simulink model "simWECS_2019a_LUT"  (R2019a)
settings: Solver=FixedStepAuto  StartTime=0.0  StopTime=40*DT  FixedStep=DT  RelTol=1e-3
values from neighbouring files (symbols this model uses):
  Cq = 0.0 0.0 0.0 0.0 0.0 0.0 0.0 0.0 0.0 0.0 0.0 0.0 0.0 0.0 0.0 0.0 0.0 0.0 0.0 0.0 0.0 0.0 0.0 0.0 0.0 0.0 0.0 0.0 0.0 0.0 0.0 0.0 0.0 0.0 0.0 0.0 0.0 0.0 0.0 0.0 0.0 0.0 0.0 0.0 0.0 0.0 0.0 0.0 0.0 0.0 0.0 0.0 0.0 0.0 0.0 0.0 0.0 0.0 0.0 0.0 0.0 0.0 0.0 0.0 0.0 0.0 0.0 0.0 0.0 0.0 0.0 0.0 0.0 0.0 0.0 0.0 0.0 0.0 0.0 0.0 0.0 0.0 0.0 0.0 0.0 0.0 0.0 0.0 0.0 0.0 0.0 0.0 0.0 0.0 0.0 0.0 0.0 0.0 0.0 0.0    [DD_test.sldd]    (also in testOutList.m = saveVarsMat.Cq)
  Ct = 0.0 0.0 0.0 0.0 0.0 0.0 0.0 0.0 0.0 0.0 0.0 0.0 0.0 0.0 0.0 0.0 0.0 0.0 0.0 0.0 0.0 0.0 0.0 0.0 0.0 0.0 0.0 0.0 0.0 0.0 0.0 0.0 0.0 0.0 0.0 0.0 0.0 0.0 0.0 0.0 0.0 0.0 0.0 0.0 0.0 0.0 0.0 0.0 0.0 0.0 0.0 0.0 0.0 0.0 0.0 0.0 0.0 0.0 0.0 0.0 0.0 0.0 0.0 0.0 0.0 0.0 0.0 0.0 0.0 0.0 0.0 0.0 0.0 0.0 0.0 0.0 0.0 0.0 0.0 0.0 0.0 0.0 0.0 0.0 0.0 0.0 0.0 0.0 0.0 0.0 0.0 0.0 0.0 0.0 0.0 0.0 0.0 0.0 0.0 0.0    [DD_test.sldd]    (also in testOutList.m = saveVarsMat.Ct)
  Drivetrain = struct    [dataDLR.m]
  DT = 0.008    [dataDLR.m]    (also in generateReport.m; initLPVParam.m; initWorkspace.m; runCalculateEvalCriteria.m)
  Lin_points : value not decoded    [DD_test.sldd]
  mu_old = zeros(2*N*nu,1)    [testCtrl.m]
  Ng = 97    [dataDLR.m]    (also in testCtrl.m)
  omegabar = interp1(Lin_points.V,Lin_points.RSpeed,Vbar,'spline')    [testCtrl.m]
  rho = 1.225    [DD_test.sldd]    (also in dataDLR.m; testOutList.m; testqLPV.m)
  tau_g = 0.01    [testCtrl.m]
  U = zeros(2*N,1)    [testCtrl.m]
  xk = Xk(nxa+1:2*nxa)    [testCtrl.m]
  Xko = kron(ones(N,1),xk)    [testCtrl.m]
undefined symbols (not defined in the file or in its folder): R, Rotor_Lambda, Rotor_Lamda, Rotor_Pitch
settings Model: ExtModeTrigMode=oneshot  ExtModeArmWhenConnect=off  Creator=Hazim Namik  LastModifiedBy=bs
settings DataIOCC: LimitDataPoints=on  SaveFormat=Array  ReturnWorkspaceOutputs=off
settings OptimizationCC: BlockReduction=off  BooleanDataType=off  LifeSpan=inf
settings DebuggingCC: SaveWithParameterizedLinksMsg=none  UnderspecifiedInitializationDetection=Classic  MergeDetectMultiDrivingBlocksExec=none  SignalResolutionControl=TryResolveAllWithWarning  SFUnexpectedBacktrackingDiag=warning  SFNoUnconditionalDefaultTransitionDiag=warning  SFExecutionAtInitializationDiag=none  ArithmeticOperatorsInVariantConditions=warning
settings HardwareCC: ProdBitPerPointer=32  ProdBitPerSizeT=32  ProdBitPerPtrDiffT=32  ProdLargestAtomicFloat=None  ProdIntDivRoundTo=Undefined  ProdEndianess=Unspecified  ProdWordSize=32  ProdHWDeviceType=32-bit Generic  TargetUnknown=on
settings ModelReferenceCC: PropagateSignalLabelsOutOfModel=off
settings SFSimCC: SimUseLocalCustomCode=off
settings RTWCC: RTWUseLocalCustomCode=off
settings CodeAppCC: StateflowObjectComments=on
settings GRTTargetCC: TargetLangStandard=C89/C90 (ANSI)  GeneratePreprocessorConditionals=Disable all
settings ConfigComp: CovMetricSettings=dw  CovHtmlReporting=on  CovSaveCumulativeToWorkspaceVar=on  CovSaveSingleToWorkspaceVar=on  CovExternalEMLEnable=off

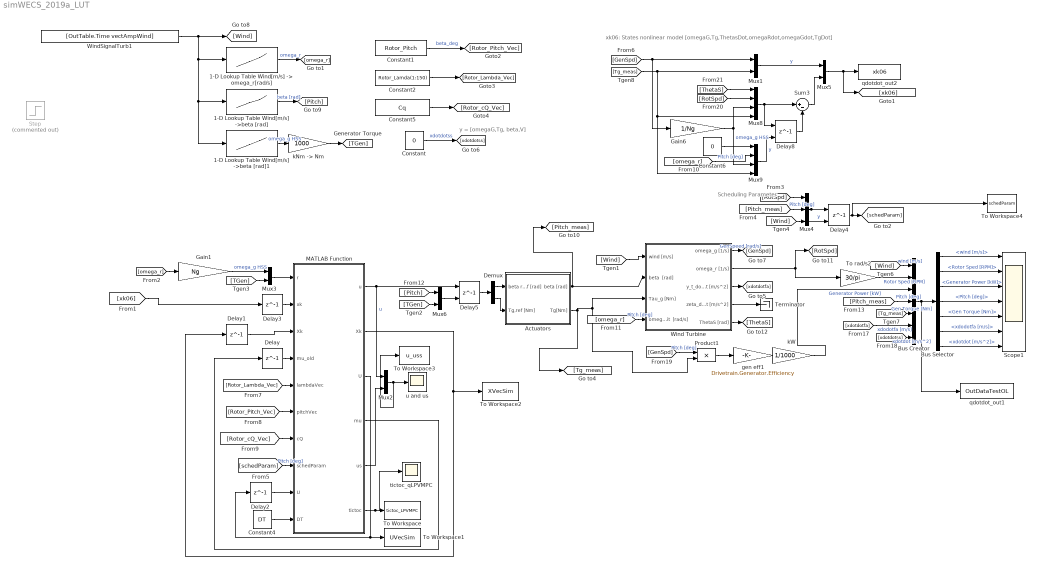
== system simWECS_2019a_LUT ==
  note: Scheduling Parameter
  note: xk06: States nonlinear model [omegaG,Tg,ThetasDot,omegaRdot,omegaGdot,TgDot]
  note: y = [omegaG,Tg, beta,V]
  "1-D Lookup Table Wind[m/s] -> omega_r[rad/s]" : Lookup_n-D  NumberOfTableDimensions=1  BreakpointsForDimension1=Lin_points.V  BreakpointsForDimension2=Rotor_Lambda  Table=Lin_points.RSpeed  InternalRulePriority=Speed  RndMeth=Simplest  InputSameDT=on
  1-D Lookup Table Wind[m/s] ->beta [rad] : Lookup_n-D  NumberOfTableDimensions=1  BreakpointsForDimension1=Lin_points.V  BreakpointsForDimension2=Rotor_Lambda  Table=Lin_points.Pitch  InternalRulePriority=Speed  RndMeth=Simplest  InputSameDT=on
  1-D Lookup Table Wind[m/s] ->beta [rad]1 : Lookup_n-D  NumberOfTableDimensions=1  BreakpointsForDimension1=Lin_points.V  BreakpointsForDimension2=Rotor_Lambda  Table=Lin_points.Torque  InternalRulePriority=Speed  RndMeth=Simplest  InputSameDT=on
  Actuators : Subsystem
  Bus Creator : BusCreator  Inputs=7
  Bus Selector : BusSelector  OutputSignals=wind [m/s],Rotor Sped [RPM],Generator Power [kW],Pitch [deg],Gen Torque [Nm],xdodotfa [m/s],xdotdot [m/s^2]
  Constant : Constant  Value=0
  Constant1 : Constant  Value=Rotor_Pitch
  Constant2 : Constant  Value=Rotor_Lamda(1:150)
  Constant4 : Constant  Value=DT
  Constant5 : Constant  Value=Cq
  Constant6 : Constant  Value=0
  Delay : Delay  DelayLength=1  InitialCondition=mu_old
  Delay1 : Delay  DelayLength=1  InitialCondition=Xko
  Delay2 : Delay  DelayLength=1  InitialCondition=U
  Delay3 : Delay  DelayLength=1  InitialCondition=xk
  Delay4 : Delay  DelayLength=1  InitialConditionSource=Input port  InitialCondition=[0,omegabar]
      settings: InputPortMap=u0,p4
  Delay5 : Delay  DelayLength=1  InitialConditionSource=Input port  InitialCondition=[0,omegabar]
      settings: InputPortMap=u0,p4
  Delay8 : Delay  DelayLength=1  InitialConditionSource=Input port  InitialCondition=[0,omegabar]
      settings: InputPortMap=u0,p4
  Demux : Demux  Outputs=2
  Gain1 : Gain  Gain=Ng
  Gain6 : Gain  Gain=1/Ng
  MATLAB Function : MATLAB Function  TreatAsAtomicUnit=on
  Mux{1..3,5..6} (5 alike) : Mux  Inputs=2
  Mux4 : Mux  Inputs=3
  Mux8 : Mux
  Mux9 : Mux
  Product1 : Product  RndMeth=Zero
  Scope1 : Scope  NumInputPorts=7
      settings: Tag=Scope
  Step : Step  Commented=on  Time=5  Before=11  After=12  SampleTime=0
  Sum3 : Sum  Inputs=|+-
  Terminator : Terminator
  To Workspace : ToWorkspace  VariableName=tictoc_LPVMPC  SaveFormat=Timeseries  SampleTime=-1
  To Workspace1 : ToWorkspace  VariableName=UVecSim  SampleTime=-1
  To Workspace2 : ToWorkspace  VariableName=XVecSim  SampleTime=-1
  To Workspace3 : ToWorkspace  VariableName=u_uss  SampleTime=-1
      settings: Save2DSignal=2-D array (concatenate along first dimension)
  To Workspace4 : ToWorkspace  VariableName=schedParam  SampleTime=-1
      settings: Save2DSignal=2-D array (concatenate along first dimension)
  To rad/s2 : Gain  Gain=30/pi
  Wind Turbine : Subsystem
  WindSignalTurb1 : FromWorkspace  VariableName=[OutTable.Time vectAmpWind]  SampleTime=DT  OutputAfterFinalValue=Holding final value
  gen eff1 : Gain  Gain=Drivetrain.Generator.Efficiency
  "kNm -> Nm" : Gain  Gain=1000
  kW : Gain  Gain=1/1000
  qdotdot_out1 : ToWorkspace  VariableName=OutDataTestOL  SampleTime=-1
  qdotdot_out2 : ToWorkspace  VariableName=xk06  SampleTime=-1
  tictoc_qLPVMPC : Scope
  u and us : Scope
  wires:
  MATLAB Function/5(us) -> Mux2/2
  1-D Lookup Table Wind[m/s] ->beta [rad]1/1 -> "kNm -> Nm"/1  "omega_g HSS"
  MATLAB Function/6(tictoc) -> tictoc_qLPVMPC/1, To Workspace/1
  "1-D Lookup Table Wind[m/s] -> omega_r[rad/s]"/1 -> [omega_r]  "omega_r"
  Delay/1 -> MATLAB Function/4(mu_old)
  Delay1/1 -> MATLAB Function/3("Xk ")
  Mux2/1 -> u and us/1, To Workspace3/1
  MATLAB Function/1(u) -> Delay5/1, Mux2/1  "u"
  MATLAB Function/4(mu) -> Delay/1
  1-D Lookup Table Wind[m/s] ->beta [rad]/1 -> [Pitch]  "beta [rad]"
  Constant2/1 -> [Rotor_Lambda_Vec]
  Constant1/1 -> [Rotor_Pitch_Vec]  "beta_deg"
  Constant5/1 -> [Rotor_cQ_Vec]
  WindSignalTurb1/1 -> 1-D Lookup Table Wind[m/s] ->beta [rad]1/1, 1-D Lookup Table Wind[m/s] ->beta [rad]/1, "1-D Lookup Table Wind[m/s] -> omega_r[rad/s]"/1, [Wind]
  "kNm -> Nm"/1 -> [TGen]
  [Rotor_Lambda_Vec] -> MATLAB Function/5(lambdaVec)
  [Rotor_Pitch_Vec] -> MATLAB Function/6(pitchVec)
  [Rotor_cQ_Vec] -> MATLAB Function/7(cQ)
  Bus Selector/6 -> Scope1/6  "<xdodotfa [m/s]>"
  Actuators/1(beta [rad]) -> [Pitch_meas], Wind Turbine/2(beta  [rad])
  To rad/s2/1 -> Bus Creator/2  "Rotor Sped [RPM]"
  Bus Selector/5 -> Scope1/5  "<Gen Torque [Nm]>"
  [GenSpd] -> Product1/1  "Pitch [deg]"
  [Tg_meas] -> Bus Creator/5  "Gen Torque [Nm]"
  [Wind] -> Wind Turbine/1(wind [m/s])
  Product1/1 -> gen eff1/1
  [xdotdotfa] -> Bus Creator/6  "xdodotfa [m/s]"
  [Pitch_meas] -> Bus Creator/4  "Pitch [deg]"
  Wind Turbine/4(zeta_dotdot [m/s^2]) -> Terminator/1
  Wind Turbine/2(omega_r [1/s]) -> To rad/s2/1, [RotSpd]
  [xdotdotss] -> Bus Creator/7  "xdotdot [m/s^2]"
  Constant/1 -> [xdotdotss]  "xdotdotss"
  Wind Turbine/1(omega_g [1/s]) -> [GenSpd]  "GenSpeed [rad/s]"
  [Wind] -> Bus Creator/1  "wind [m/s]"
  kW/1 -> Bus Creator/3  "Generator Power [kW]"
  Actuators/2(Tg[Nm]) -> [Tg_meas], Product1/2, Wind Turbine/3(Tau_g [Nm])
  Bus Creator/1 -> Bus Selector/1, qdotdot_out1/1
  Wind Turbine/3(y_t_dotdot [m/s^2]) -> [xdotdotfa]
  gen eff1/1 -> kW/1
  Wind Turbine/5(ThetaS [rad]) -> [ThetaS]
  Bus Selector/7 -> Scope1/7  "<xdotdot [m/s^2]>"
  Bus Selector/4 -> Scope1/4  "<Pitch [deg]>"
  Bus Selector/3 -> Scope1/3  "<Generator Power [kW]>"
  Bus Selector/2 -> Scope1/2  "<Rotor Sped [RPM]>"
  Bus Selector/1 -> Scope1/1  "<wind [m/s]>"
  [xk06] -> Delay3/1
  Delay2/1 -> MATLAB Function/9("U ")
  MATLAB Function/3(U) -> To Workspace1/1, Delay2/1
  [RotSpd] -> Mux4/1
  [Pitch_meas] -> Mux4/2  "Pitch [deg]"
  [Wind] -> Mux4/3
  [schedParam] -> MATLAB Function/8(schedParam)  "Pitch [deg]"
  Constant4/1 -> MATLAB Function/10(DT)
  Mux3/1 -> MATLAB Function/1(r)
  [omega_r] -> Gain1/1
  [TGen] -> Mux3/2
  Delay3/1 -> MATLAB Function/2(xk)
  MATLAB Function/2(Xk) -> To Workspace2/1, Delay1/1
  Demux/2 -> Actuators/2(Tg,ref [Nm])
  Demux/1 -> Actuators/1(beta ref [rad])
  [omega_r] -> Mux9/2  "Pitch [deg]"
  Constant6/1 -> Mux9/1
  Delay8/1 -> Sum3/2
  [ThetaS] -> Mux8/1
  Mux8/1 -> Sum3/1, Delay8/1
  [Tg_meas] -> Mux9/4, Mux8/4, Mux1/2
  Mux1/1 -> Mux5/1  "y"
  Mux9/1 -> Delay8/2  "y"
  [GenSpd] -> Gain6/1, Mux1/1
  [RotSpd] -> Mux8/2
  Gain6/1 -> Mux8/3, Mux9/3  "omega_g HSS"
  Mux5/1 -> [xk06], qdotdot_out2/1
  Sum3/1 -> Mux5/2
  Gain1/1 -> Mux3/1  "omega_g HSS"
  Delay4/1 -> To Workspace4/1, [schedParam]
  Mux4/1 -> Delay4/2, Delay4/1  "y"
  [Pitch] -> Mux6/1
  [TGen] -> Mux6/2
  Mux6/1 -> Delay5/2
  Delay5/1 -> Demux/1
  [omega_r] -> Wind Turbine/4(omega_r_init  [rad/s])  "Pitch [deg]"

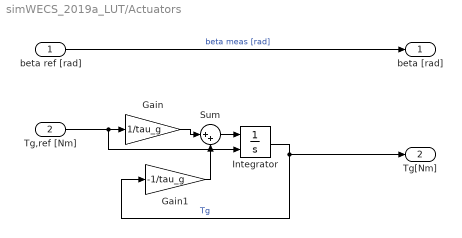
== system simWECS_2019a_LUT/Actuators ==
  beta ref [rad] : Inport
  Tg,ref [Nm] : Inport  Port=2
  Gain : Gain  Gain=1/tau_g
  Gain1 : Gain  Gain=-1/tau_g
  Integrator : Integrator  InitialConditionSource=external
  Sum : Sum  Inputs=|++
  beta [rad] : Outport
  Tg[Nm] : Outport  Port=2
  wires:
  Tg,ref [Nm]/1 -> Gain/1, Integrator/2
  Integrator/1 -> Tg[Nm]/1, Gain1/1  "Tg"
  beta ref [rad]/1 -> beta [rad]/1  "beta meas [rad]"
  Gain/1 -> Sum/1
  Sum/1 -> Integrator/1
  Gain1/1 -> Sum/2

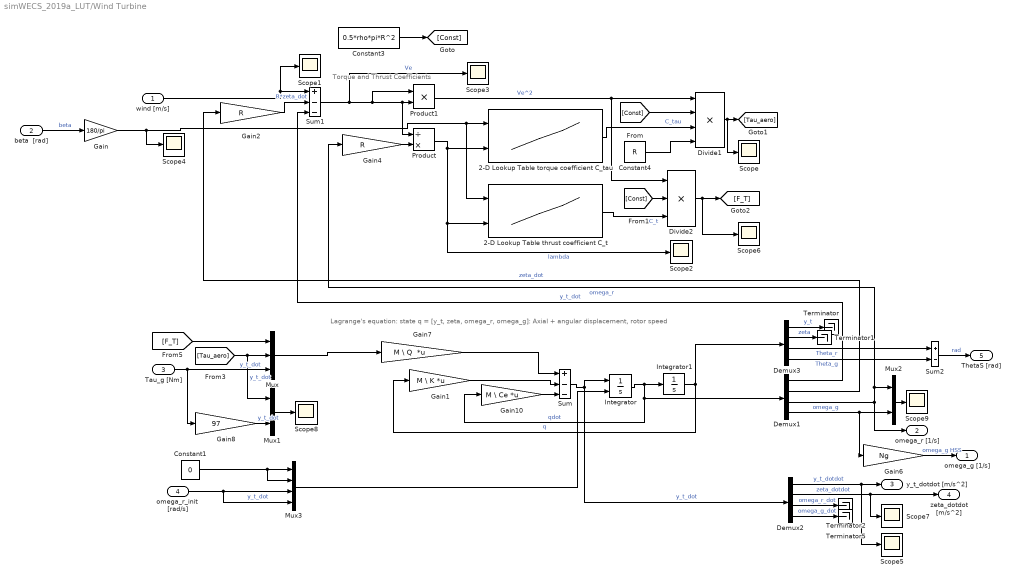
== system simWECS_2019a_LUT/Wind Turbine ==
  note: Torque and Thrust Coefficients
  note: Lagrange's equation: state q = [y_t, zeta, omega_r, omega_g]: Axial + angular displacement, rotor speed
  wind [m/s] : Inport
  beta  [rad] : Inport  Port=2
  Tau_g [Nm] : Inport  Port=3
  omega_r_init  [rad/s] : Inport  Port=4
  2-D Lookup Table thrust coefficient C_t : Lookup_n-D  BreakpointsForDimension1=Rotor_Pitch  BreakpointsForDimension2=Rotor_Lambda  Table=Ct  InternalRulePriority=Speed  RndMeth=Simplest  InputSameDT=on
  2-D Lookup Table torque coefficient C_tau : Lookup_n-D  BreakpointsForDimension1=Rotor_Pitch  BreakpointsForDimension2=Rotor_Lambda  Table=Cq  InternalRulePriority=Speed  RndMeth=Simplest  InputSameDT=on
  Constant1 : Constant  Value=0
  Constant3 : Constant  Value=0.5*rho*pi*R^2
  Constant4 : Constant  Value=R
  Demux1 : Demux
  Demux2 : Demux
  Demux3 : Demux
  Divide1 : Product  Inputs=****
  Divide2 : Product  Inputs=***
  Gain : Gain  Gain=180/pi
  Gain1 : Gain  Gain=M \ K  Multiplication=Matrix(K*u)
  Gain10 : Gain  Gain=M \ Ce  Multiplication=Matrix(K*u)
  Gain2 : Gain  Gain=R
  Gain4 : Gain  Gain=R
  Gain6 : Gain  Gain=Ng
  Gain7 : Gain  Gain=M \ Q  Multiplication=Matrix(K*u)
  Gain8 : Gain  Gain=97
  Integrator : Integrator  InitialConditionSource=external  InitialCondition=[0,0,0.5, 0.5]
  Integrator1 : Integrator  InitialCondition=[0,0,0,0]
  Mux : Mux  Inputs=3
  Mux1 : Mux  Inputs=2
  Mux2 : Mux  Inputs=2
  Mux3 : Mux
  Product : Product  Inputs=/*
  Product1 : Product  Inputs=**
  Scope{,1..9} (10 alike) : Scope
  Sum : Sum  Inputs=+--
  Sum1 : Sum  Inputs=+--
  Sum2 : Sum  Inputs=+-
  Terminator{,1..2,5} (4 alike) : Terminator
  omega_g [1/s] : Outport
  omega_r [1/s] : Outport  Port=2
  y_t_dotdot [m/s^2] : Outport  Port=3
  zeta_dotdot [m/s^2] : Outport  Port=4
  ThetaS [rad] : Outport  Port=5
  wires:
  Constant4/1 -> Divide1/4
  Sum1/1 -> Scope3/1, Product1/1, Product1/2, Product/1  "Ve"
  wind [m/s]/1 -> Sum1/1, Scope1/1
  Gain4/1 -> Product/2
  Divide2/1 -> [F_T], Scope6/1
  2-D Lookup Table thrust coefficient C_t/1 -> Divide2/3  "C_t"
  Divide1/1 -> Scope/1, [Tau_aero]
  [Const] -> Divide1/2
  [Const] -> Divide2/2
  2-D Lookup Table torque coefficient C_tau/1 -> Divide1/3  "C_tau"
  Gain1/1 -> Sum/2
  Gain7/1 -> Sum/1
  Mux/1 -> Gain7/1
  Integrator1/1 -> Gain1/1, Demux3/1  "q"
  [F_T] -> Mux/1
  Demux1/1 -> Sum1/3  "y_t_dot"
  Demux1/2 -> Gain2/1  "zeta_dot"
  Demux1/3 -> Gain4/1, Mux2/1, omega_r [1/s]/1  "omega_r"
  Demux1/4 -> Gain6/1, Mux2/2  "omega_g"
  Gain2/1 -> Sum1/2  "R*zeta_dot"
  Demux2/1 -> Scope5/1, y_t_dotdot [m/s^2]/1  "y_t_dotdot"
  Demux2/2 -> zeta_dotdot [m/s^2]/1, Scope7/1  "zeta_dotdot"
  Demux2/4 -> Terminator5/1  "omega_g_dot"
  Demux2/3 -> Terminator2/1  "omega_r_dot"
  beta  [rad]/1 -> Gain/1  "beta"
  Product/1 -> 2-D Lookup Table thrust coefficient C_t/2, Scope2/1, 2-D Lookup Table torque coefficient C_tau/2  "lambda"
  Product1/1 -> Divide1/1, Divide2/1  "Ve^2"
  Integrator/1 -> Gain10/1, Demux1/1, Integrator1/1  "qdot"
  Demux3/1 -> Terminator/1  "y_t"
  Demux3/2 -> Terminator1/1  "zeta"
  Demux3/3 -> Sum2/1  "Theta_r"
  Demux3/4 -> Sum2/2  "Theta_g"
  Gain10/1 -> Sum/3
  Gain6/1 -> omega_g [1/s]/1  "omega_g HSS"
  Constant3/1 -> [Const]
  [Tau_aero] -> Mux1/1, Mux/2  "y_t_dot"
  Mux1/1 -> Scope8/1
  Tau_g [Nm]/1 -> Gain8/1, Mux/3  "y_t_dot"
  Mux2/1 -> Scope9/1
  Sum/1 -> Demux2/1, Integrator/1  "y_t_dot"
  Gain8/1 -> Mux1/2  "y_t_dot"
  Sum2/1 -> ThetaS [rad]/1  "rad"
  Gain/1 -> 2-D Lookup Table thrust coefficient C_t/1, 2-D Lookup Table torque coefficient C_tau/1, Scope4/1
  omega_r_init  [rad/s]/1 -> Mux3/4, Mux3/3  "y_t_dot"
  Constant1/1 -> Mux3/2, Mux3/1
  Mux3/1 -> Integrator/2

== matlab function simWECS_2019a_LUT/MATLAB Function ==
  settings: updateMethod=DISCRETE
  data: r input; u output; xk input; Xk input; mu_old input; lambdaVec input; pitchVec input; cQ input; schedParam input; U input; DT input; Xk output; U output; mu output; us output; tictoc output
function [u,Xk,U,mu,us,tictoc]= qLPVMPC_WECS(r,xk,Xk,mu_old,lambdaVec,pitchVec,cQ,schedParam,U,DT)
% MATLAB_Function calculates controller output u. It turns the QP into a 
% linear complementarity problem (LCP) and solves it with Lemke's algorithm.
%
% Inputs: * r: reference
%         * xk: quasiLPV KF state estimates
%         * Xk: Xko(= L*xk+S*U) delayed by one sample timestep
%         * mu_old: mu delayed by one sample timestep
%         * lambdaVec: lambda vector for cQ LUT 
%         * pitchVec: pitch vector for cQ LUT 
%         * cQ: torque coefficients LUT matrix
%         * schedParam: current values [omegaR, beta, V]
%         * U: U (from Xko = L*xk+S*U) delayed by one sample timestep
%
% Outputs: * u: controller output at current time step
%          * Xko: Future state trajectory (L*xk+S*U)
%          * U: Future input trajectory 
%          * mu: Result Lemke's algorithm/LCP: M mu +q >=0, mu>=0, mu'(Mmu+q)=0
%          * us: xuss(end) from xuss = [eye(4)-Ass -Bss;[1 0 0 0] 0]\[Bss*d;1]
%          * tictoc: tic-toc result

% Pablo S.G. Cisneros, Herbert Werner, ICS TUHH

%#codegen
coder.extrinsic('tic');
coder.extrinsic('toc');
tictoc = 0;
tic

%% Init N, Q, R
N = 40;
q_ = [1000 1 1 1 100 1]; %q_ = [100 1000 1 0.01 0]; 7.351e+02 1.000e+00 1.938e+09 1.625e+08 1.491e+08 1.657e+03
R_ = kron(eye(N),diag([1000,1])); %R_ = 1000*eye(N); 
p = 100*q_; %P = 1000*diag(q_);

Ulim = repmat([8 * pi/180, 20000]',2*N,1); %rate constraints 
Ng = 97;

Control_Pitch_Max = 90 /180 * pi;
Control_Pitch_Min = -2 /180 * pi;
Control_Torque_Limit = 47403;
Control_Torque_Min = 200;
schedParam(2) = min(max(schedParam(2), Control_Pitch_Min),Control_Pitch_Max);

isBetaState = 0;
nx = 4 + isBetaState; % number states plant: ThetaS,omegaR,omegaG,Tg
ny = 2 + isBetaState; % number of outputs plant omegaG,Tg
nxA = nx +ny; %number states augmented plant 
nu = 2; % plant inputs: Tg_ref, beta_ref

%% Shift Xk
Xk(1:end-nxA) = Xk(nxA+1:end); 
%Xk(1:nxA)

%% Create augmented system: C matrix orig. mdl, A, B matrices augmented
C1 = [zeros(ny,nx-ny), diag([Ng, ones(1,ny-1)])];

%% Calculate input u_dot_s = 0  and steady state x = r
us = [0;0]; %xuss(nxA+1:nxA+2); % xuss = [eye(size(Ass))-Ass -Bss;[1 0 0 0] 0] \ [Bss*d;reference];

iterations = 1; % omega_ref(Vest), Tg_ref(Vest)
refVec = zeros(nxA,1);
refVec(1:2) = r;
ref = repmat(refVec,N,1); %ref = kron(ones(N,1),[r; 0; 0; 0;0]);

for i = 1:iterations
    [L,S,H,g] = HSqLd_WT(N,q_,R_,p,xk,Xk,DT,ref,us,lambdaVec,pitchVec,cQ,C1,schedParam,U);
    
    %% %%%%%%Turn QP into LCP and solve it%%%%%%%%%
    Ac_ = [-eye(N*nu);eye(N*nu)];
    bc_ = - Ulim;
    Hi = eye(size(H,1))/H;
    M = Ac_*Hi*Ac_';
    q = -Ac_*Hi*g - bc_;
 
    mu = lemke(M,q,mu_old);
 
    U = Hi*(Ac_'*mu-g);
    U(isnan(U)) = 0;
    
    %% %%%%%%%%%%%%%%%%%%%%%%%%%%%%%%%%%%%%%%%%%%%%    
    Xk = L*xk+S*U;
end

u =  [min( max(U(1) + schedParam(2), Control_Pitch_Min),Control_Pitch_Max),... % pitch
min(max(U(2) + Xk(2), Control_Torque_Min),Control_Torque_Limit)]'; % torque

tictoc = toc;
